simulink model "utfyllende_model"  (R2025b)
settings: Solver=VariableStepAuto  StartTime=0.0  StopTime=0.1  RelTol=1e-3
undefined symbols (not defined in the file or in its folder): B_m, I_annet, J_m, K, k_Q, L_m, R_b, R_l, R_m, V_b
libraries: simulink x1, slpidlib x1
settings Model: Creator=vikin  LastModifiedBy=vikin

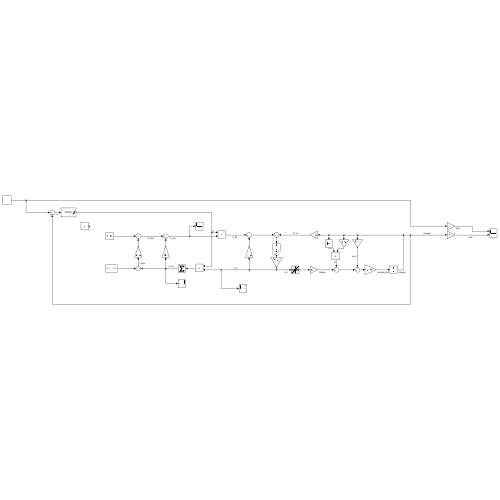
[thumbnail: Simulink's stored preview of the top-level diagram]
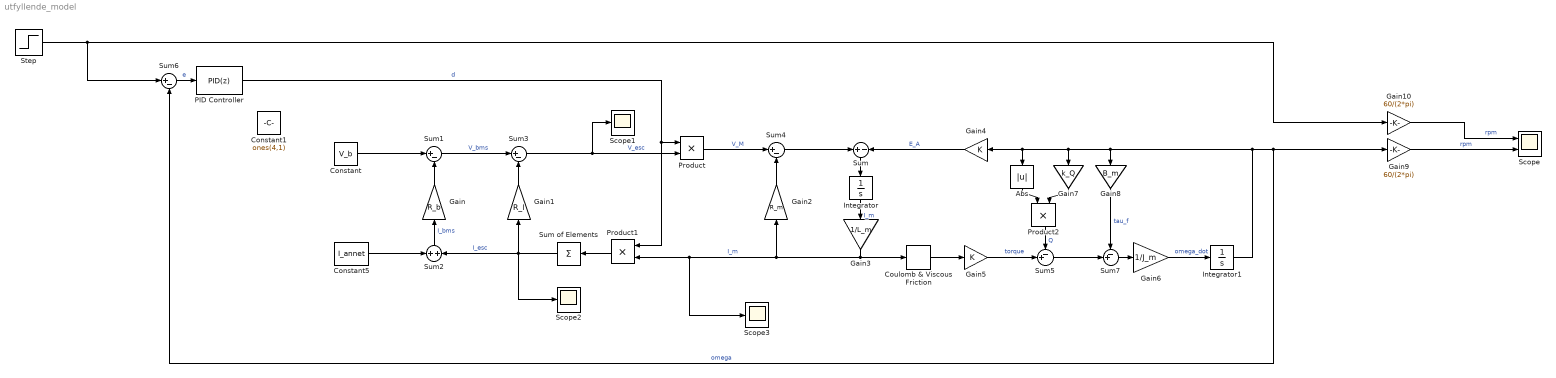
== system utfyllende_model ==
  Abs : Abs  SaturateOnIntegerOverflow=off
  Constant : Constant  Value=V_b
  Constant1 : Constant  Value=ones(4,1)
  Constant5 : Constant  Value=I_annet
  Coulomb & Viscous Friction : simulink/Discontinuities/Coulomb & Viscous Friction  offset=I_0  gain=1
  Gain : Gain  Gain=R_b
  Gain1 : Gain  Gain=R_l
  Gain10 : Gain  Gain=60/(2*pi)
  Gain2 : Gain  Gain=R_m
  Gain3 : Gain  Gain=1/L_m
  Gain4 : Gain  Gain=K
  Gain5 : Gain  Gain=K
  Gain6 : Gain  Gain=1/J_m
  Gain7 : Gain  Gain=k_Q
  Gain8 : Gain  Gain=B_m
  Gain9 : Gain  Gain=60/(2*pi)
  Integrator : Integrator  InitialCondition=zeros(4,1)
  Integrator1 : Integrator  InitialCondition=zeros(4,1)
  PID Controller : slpidlib/PID Controller  Controller=PID  Form=Parallel  TimeDomain=Discrete-time  UseExternalTs=off  SampleTime=0.0001  IntegratorMethod=Forward Euler  FilterMethod=Forward Euler  ControllerParametersSource=internal  P=0.002  I=4  UseKiTs=off  D=0.01  UseExternalDerivativeSource=off  N=1  UseFilter=on  TunerSelectOption=Transfer Function Based (PID Tuner App)  InitialConditionSource=internal  InitialConditionForIntegrator=0  InitialConditionForFilter=0  DifferentiatorICPrevScaledInput=0  ExternalReset=none  TrackingMode=off  Kt=1  LimitOutput=on  SatLimitsSource=internal  UpperSaturationLimit=1  LowerSaturationLimit=-1  LinearizeAsGain=on  AntiWindupMode=clamping  Kb=1  LimitIntegrator=off  UpperIntegratorSaturationLimit=inf  LowerIntegratorSaturationLimit=-inf  POutMin=[]  POutMax=[]  IOutMin=[]  IOutMax=[]  DOutMin=[]  DOutMax=[]  NOutMin=[]  NOutMax=[]  SumOutMin=[]  SumOutMax=[]  SaturationOutMin=[]  SaturationOutMax=[]  PParamMin=[]  PParamMax=[]  IParamMin=[]  IParamMax=[]  DParamMin=[]  DParamMax=[]  NParamMin=[]  NParamMax=[]  KbParamMin=[]  KbParamMax=[]  KtParamMin=[]  KtParamMax=[]  KbOutMin=[]  KbOutMax=[]  KtOutMin=[]  KtOutMax=[]  IntegratorOutMin=[]  IntegratorOutMax=[]  FilterOutMin=[]  FilterOutMax=[]  SumI1OutMin=[]  SumI1OutMax=[]  SumI2OutMin=[]  SumI2OutMax=[]  SumI3OutMin=[]  SumI3OutMax=[]  SumI4OutMin=[]  SumI4OutMax=[]  SumDOutMin=[]  SumDOutMax=[]  DifferentiatorOutMin=[]  DifferentiatorOutMax=[]  FilterDiffOutCoefMin=[]  FilterDiffOutCoefMax=[]  ReciprocalOutMin=[]  ReciprocalOutMax=[]  SumDenOutMin=[]  SumDenOutMax=[]  SumNumOutMin=[]  SumNumOutMax=[]  DivideOutMin=[]  DivideOutMax=[]  UdiffTsProdOutMin=[]  UdiffTsProdOutMax=[]  NTsProdOutMin=[]  NTsProdOutMax=[]  UintegralTsProdOutMin=[]  UintegralTsProdOutMax=[]  UngainTsProdOutMin=[]  UngainTsProdOutMax=[]  ClampingZeroOutDataTypeStr=Inherit: Inherit via back propagation  ClampingZeroOutMin=[]  ClampingZeroOutMax=[]  FilterDenConstantOutDataTypeStr=Inherit: Inherit via back propagation  FilterDenConstantOutMin=[]  FilterDenConstantOutMax=[]  PCopyOutDataTypeStr=Inherit: Inherit via back propagation  PCopyOutMin=[]  PCopyOutMax=[]  NCopyOutDataTypeStr=Inherit: Inherit via back propagation  NCopyOutMin=[]  NCopyOutMax=[]  IntegratorContinuousStateAttributes=''  IntegratorStateMustResolveToSignalObject=off  IntegratorRTWStateStorageClass=Auto  FilterContinuousStateAttributes=''  FilterStateMustResolveToSignalObject=off  FilterRTWStateStorageClass=Auto  ParallelPVariant=InternalParameters  IdealPVariant=Disabled  IVariant=InternalParameters  DVariant=InternalParameters  IntegratorVariant=Discrete  SatVariant=Enabled  AWVariant=DiscClampingParallel  PCopyVariant=Disabled  TRVariant=Disabled  FdbkBlocksVariant=Forward  IdealPFdbkVariant=Disabled  SatFdbkVariant=Disabled  DerivativeFilterVariant=ForwardEulerFilter  NVariant=InternalParameters  NCopyVariant=Disabled  FilterICVariant=InternalICsFilter  IntegratorICVariant=InternalICs  ExternalResetVariant=Disabled  TRSumVariant=Passthrough  SumFdbkVariant=Disabled  SumVariant=Sum_PID  TsampFilterVariant=InternalTs  TsampNgainVariant=Passthrough  TsampIntegralVariant=Disabled_SignalSpec  ExternalSaturationOutDataTypeStr=Inherit: Same as second input  DerivativeSourceVariant=ErrorSignal  PreIntVariant=InternalPreInt
  Product : Product
  Product1 : Product
  Product2 : Product
  Scope : Scope  NumInputPorts=2
      settings: ActiveDisplayYMinimum=-270.12094369332885  ActiveDisplayYMaximum=3991.2760685121425
  Scope1 : Scope
      settings: ActiveDisplayYMinimum=10.001520884778081  ActiveDisplayYMaximum=16.660942123913546
  Scope2 : Scope
      settings: ActiveDisplayYMinimum=-64.592462661468431  ActiveDisplayYMaximum=581.332163953216  DataLoggingVariableName=ScopeData2
  Scope3 : Scope
      settings: ActiveDisplayYMinimum=-16.148115665367108  ActiveDisplayYMaximum=145.333040988304  DataLoggingVariableName=ScopeData3
  Step : Step  Time=0.05  Before=zeros(4,1)  After=ones(4,1)*340  SampleTime=0
  Sum : Sum  Inputs=+|-
  Sum of Elements : Sum  Inputs=+
  Sum{1,3..4,6} (4 alike) : Sum  Inputs=|+-
  Sum2 : Sum  Inputs=+|+
  Sum5 : Sum  Inputs=-+|
  Sum7 : Sum  Inputs=-+|
  wires:
  Constant/1 -> Sum1/1
  Sum1/1 -> Sum3/1  "V_bms"
  Constant5/1 -> Sum2/1
  Step/1 -> Sum6/1, Gain10/1
  Gain/1 -> Sum1/2
  Sum2/1 -> Gain/1  "I_bms"
  Gain1/1 -> Sum3/2
  Sum of Elements/1 -> Scope2/1, Gain1/1, Sum2/2  "I_esc"
  Product/1 -> Sum4/1  "V_M"
  Gain2/1 -> Sum4/2
  Product1/1 -> Sum of Elements/1
  PID Controller/1 -> Product/1, Product1/1  "d"
  Sum3/1 -> Product/2, Scope1/1  "V_esc"
  Sum4/1 -> Sum/1
  Integrator/1 -> Gain3/1  "I_m"
  Sum/1 -> Integrator/1
  Sum6/1 -> PID Controller/1  "e"
  Integrator1/1 -> Gain8/1, Gain4/1, Abs/1, Gain7/1, Sum6/2, Gain9/1  "omega"
  Gain3/1 -> Coulomb & Viscous Friction/1, Gain2/1, Scope3/1, Product1/2  "I_m"
  Gain4/1 -> Sum/2  "E_A"
  Gain7/1 -> Product2/2
  Product2/1 -> Sum5/1  "Q"
  Abs/1 -> Product2/1
  Sum5/1 -> Sum7/2
  Gain6/1 -> Integrator1/1  "omega_dot"
  Gain5/1 -> Sum5/2  "torque"
  Coulomb & Viscous Friction/1 -> Gain5/1
  Sum7/1 -> Gain6/1
  Gain8/1 -> Sum7/1  "tau_f"
  Gain9/1 -> Scope/2  "rpm"
  Gain10/1 -> Scope/1  "rpm"
